simulink model "UAV_GuidanceWaypointScenario"  (R2026a)
settings: Solver=ode45  StopTime=60  MaxStep=0.01
PreLoadFcn:
  | setup_uav_scenario;  % scene must exist before the Scenario blocks initialise on load
InitFcn:
  | setup_uav_scenario;  % recreate the uavScenario handle object before each run
model workspace (MAT data in the model file):
  ctrl.mass = 0.1
  ctrl.g = 9.81
  ctrl.Kp_pos = 0.8
  ctrl.vMaxXY = 3
  ctrl.vMaxZ = 1.5
  ctrl.Kv = 2
  ctrl.tiltMax = 0.35
  ctrl.thrustMax = 2
  ctrl.Kyaw = 2
  ctrl.yawRateMax = 1
  gravityNED = 9.81
  hoverThrust = 0.981
  lookaheadDist = 3
  transitionRadius = 1.5
  uavMass = 0.1
  waypoints = [0  0  -5; 20  0  -5; 20  20  -5; 0  20  -5; 0  0  -5]
values from neighbouring files (symbols this model uses):
  lidarSampleTime = 0.1    [setup_uav_scenario.m]
  scenarioSampleTime = 0.1    [setup_uav_scenario.m]
undefined symbols (not defined in the file or in its folder): Lidar, UAV
libraries: uavsimlib x4, uavalgslib x2, robotcorelib x1
settings Model: Creator=PattarapolSangaroon  LastModifiedBy=PattarapolSangaroon

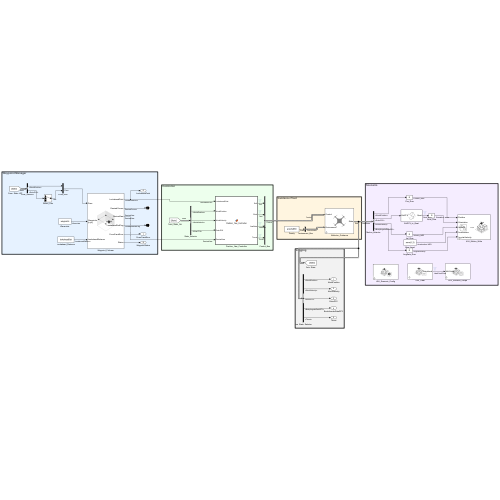
[thumbnail: Simulink's stored preview of the top-level diagram]
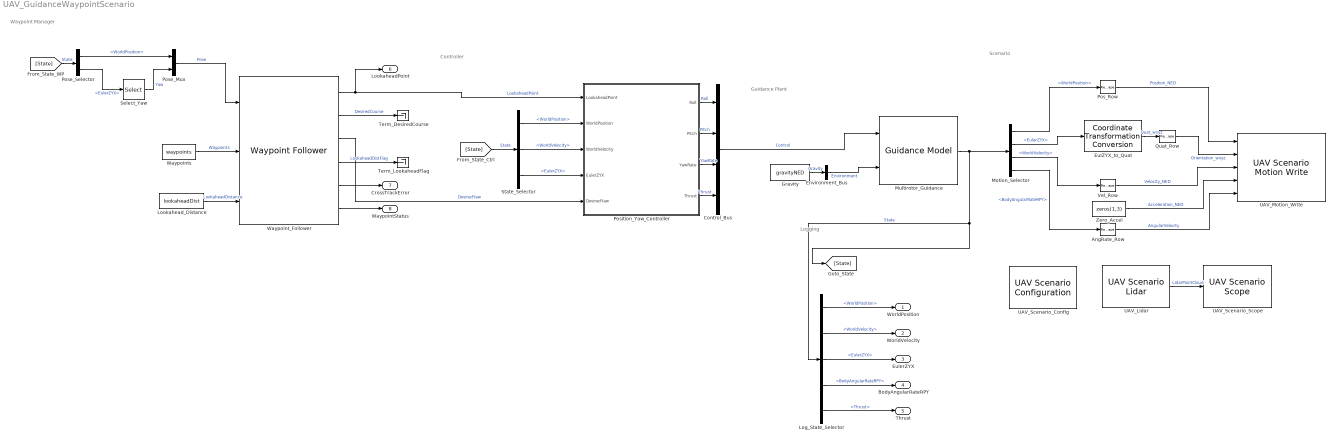
== system UAV_GuidanceWaypointScenario ==
  note: Waypoint Manager
  note: Controller
  note: Guidance Plant
  note: Scenario
  note: Logging
  AngRate_Row : Reshape  OutputDimensionality=Customize  OutputDimensions=[1 3]
  Control_Bus : BusCreator  Inputs=4  OutDataTypeStr=Bus: MultirotorGuidanceControlBus  NonVirtualBus=on
  Environment_Bus : BusCreator  Inputs=1  OutDataTypeStr=Bus: MultirotorGuidanceEnvironmentBus  NonVirtualBus=on
  EulZYX_to_Quat : robotcorelib/Coordinate Transformation Conversion  InputRepresentation=Euler Angles  InputEulerSequence=ZYX  ShowTrVecInputPort=on  OutputRepresentation=Quaternion  OutputEulerSequence=ZYX  ShowTrVecOutputPort=on  SimulateUsing=Code generation
      settings: LibrarySourceBlock=uavutilslib/Coordinate Transformation Conversion
  Gravity : Constant  Value=gravityNED
  Log_State_Selector : BusSelector  OutputSignals=WorldPosition,WorldVelocity,EulerZYX,BodyAngularRateRPY,Thrust
  Lookahead_Distance : Constant  Value=lookaheadDist
  Motion_Selector : BusSelector  OutputSignals=WorldPosition,EulerZYX,WorldVelocity,BodyAngularRateRPY
  Multirotor_Guidance : uavalgslib/Guidance Model  ModelType=MultirotorGuidance  NumInstances=1  SpecifiedDataType=double  SimulateUsing=Code generation  InitialWorldPositionMultirotor=[0; 0; 0]  InitialWorldVelocityMultirotor=[0; 0; 0]  InitialEulerZYXMultirotor=[0; 0; 0]  InitialBodyAngularRateRPYMultirotor=[0; 0; 0]  InitialThrustMultirotor=hoverThrust  InitialNorthFixedWing=0  InitialEastFixedWing=0  InitialHeightFixedWing=0  InitialAirSpeedFixedWing=0  InitialHeadingAngleFixedWing=0  InitialFlightPathAngleFixedWing=0  InitialRollAngleFixedWing=0  InitialRollAngleRateFixedWing=0  PDRollMultirotor=[3402.97,116.67]  PDPitchMultirotor=[3402.97, 116.67]  PYawRateMultirotor=1950  PThrustMultirotor=3900  MassMultirotor=uavMass  PHeightFixedWing=3.9  PHeadingAngleFixedWing=3.9  PFlightPathAngleFixedWing=39  PDRollFixedWing=[3402.97, 116.67]  PAirSpeedFixedWing=1  FlightPathAngleLimitsFixedWing=[-pi/2, pi/2]  StateBusName='MultirotorGuidanceStateBus'  ControlBusName='MultirotorGuidanceControlBus'  EnvironmentBusName='MultirotorGuidanceEnvironmentBus'  DataType=double
  Pos_Row : Reshape  OutputDimensionality=Customize  OutputDimensions=[1 3]
  Pose_Mux : Mux  Inputs=2
  Pose_Selector : BusSelector  OutputSignals=WorldPosition,EulerZYX
  Position_Yaw_Controller : MATLAB Function  TreatAsAtomicUnit=on
  Quat_Row : Reshape  OutputDimensionality=Customize  OutputDimensions=[1 4]
  Select_Yaw : Selector  InputPortWidth=3  IndexOptions=Index vector (dialog)  Indices=1  OutputSizes=1
  State_Selector : BusSelector  OutputSignals=WorldPosition,WorldVelocity,EulerZYX
  Term_DesiredCourse : Terminator
  Term_LookaheadFlag : Terminator
  UAV_Lidar : uavsimlib/UAV Scenario Lidar  Priority=3  SensorName=UAV/Lidar  MaxRange=30  RangeAccuracy=0.02  AzimuthLimits=[-180 180]  AzimuthResolution=2  ElevationLimits=[-20 20]  ElevationResolution=2  HasNoise=off  HasOrganizedOutput=off  SampleTime=lidarSampleTime
  UAV_Motion_Write : uavsimlib/UAV Scenario Motion Write  Priority=2  PlatName='UAV'  ReferenceFrame=NED
  UAV_Scenario_Config : uavsimlib/UAV Scenario Configuration  Priority=1  UAVScenarioObject=uavScene  SampleTime=scenarioSampleTime  UpdateParam=false  SensorMotionBusName='SensorMotionBus'  PlatformMotionBusName='PlatformMotionBus'  ScenarioMotionBusName='ScenarioMotionBus'  ScenarioMotionSignalName='ScenarioMotions'
  UAV_Scenario_Scope : uavsimlib/UAV Scenario Scope  Priority=4  SensorNameTable={'UAV/Lidar','on'}  SampleTime=lidarSampleTime
  Vel_Row : Reshape  OutputDimensionality=Customize  OutputDimensions=[1 3]
  Waypoint_Follower : uavalgslib/Waypoint Follower  UAVType=multirotor  StartFrom=first  TransitionRadiusSource=internal  TransitionRadius=transitionRadius  MinLookaheadDistance=0.1  HoverAtLastWaypoint=on  InterpolateYaw=on  YawInput=off  ShowCrossTrackErrorOutput=on  ShowStatusOutput=on  ShowWaypointIndexOutput=off  SimulateUsing=Code generation
  Waypoints : Constant  Value=waypoints
  Zero_Accel : Constant  Value=zeros(1,3)
  WorldPosition : Outport
  WorldVelocity : Outport  Port=2
  EulerZYX : Outport  Port=3
  BodyAngularRateRPY : Outport  Port=4
  Thrust : Outport  Port=5
  LookaheadPoint : Outport  Port=6
  CrossTrackError : Outport  Port=7
  WaypointStatus : Outport  Port=8
  wires:
  Log_State_Selector/4 -> BodyAngularRateRPY/1  "<BodyAngularRateRPY>"
  Log_State_Selector/3 -> EulerZYX/1  "<EulerZYX>"
  Log_State_Selector/2 -> WorldVelocity/1  "<WorldVelocity>"
  Log_State_Selector/1 -> WorldPosition/1  "<WorldPosition>"
  Log_State_Selector/5 -> Thrust/1  "<Thrust>"
  [State] -> Pose_Selector/1  "State"
  Pose_Selector/1 -> Pose_Mux/1  "<WorldPosition>"
  Pose_Selector/2 -> Select_Yaw/1  "<EulerZYX>"
  Select_Yaw/1 -> Pose_Mux/2  "Yaw"
  Pose_Mux/1 -> Waypoint_Follower/1  "Pose"
  Waypoints/1 -> Waypoint_Follower/2  "Waypoints"
  Lookahead_Distance/1 -> Waypoint_Follower/3  "LookaheadDistance"
  Waypoint_Follower/1 -> Position_Yaw_Controller/1(LookaheadPoint), LookaheadPoint/1  "LookaheadPoint"
  Waypoint_Follower/2 -> Term_DesiredCourse/1  "DesiredCourse"
  Waypoint_Follower/3 -> Position_Yaw_Controller/5(DesiredYaw)  "DesiredYaw"
  Waypoint_Follower/4 -> Term_LookaheadFlag/1  "LookaheadDistFlag"
  Waypoint_Follower/5 -> CrossTrackError/1
  Waypoint_Follower/6 -> WaypointStatus/1
  [State] -> State_Selector/1  "State"
  State_Selector/1 -> Position_Yaw_Controller/2(WorldPosition)  "<WorldPosition>"
  State_Selector/2 -> Position_Yaw_Controller/3(WorldVelocity)  "<WorldVelocity>"
  State_Selector/3 -> Position_Yaw_Controller/4(EulerZYX)  "<EulerZYX>"
  Position_Yaw_Controller/1(Roll) -> Control_Bus/1  "Roll"
  Position_Yaw_Controller/2(Pitch) -> Control_Bus/2  "Pitch"
  Position_Yaw_Controller/3(YawRate) -> Control_Bus/3  "YawRate"
  Position_Yaw_Controller/4(Thrust) -> Control_Bus/4  "Thrust"
  Control_Bus/1 -> Multirotor_Guidance/1  "Control"
  Gravity/1 -> Environment_Bus/1  "Gravity"
  Environment_Bus/1 -> Multirotor_Guidance/2  "Environment"
  Multirotor_Guidance/1 -> [State], Log_State_Selector/1, Motion_Selector/1  "State"
  Motion_Selector/1 -> Pos_Row/1  "<WorldPosition>"
  Motion_Selector/2 -> EulZYX_to_Quat/1  "<EulerZYX>"
  EulZYX_to_Quat/1 -> Quat_Row/1  "Quat_wxyz"
  Motion_Selector/3 -> Vel_Row/1  "<WorldVelocity>"
  Motion_Selector/4 -> AngRate_Row/1  "<BodyAngularRateRPY>"
  Pos_Row/1 -> UAV_Motion_Write/1  "Position_NED"
  Quat_Row/1 -> UAV_Motion_Write/2  "Orientation_wxyz"
  Vel_Row/1 -> UAV_Motion_Write/3  "Velocity_NED"
  Zero_Accel/1 -> UAV_Motion_Write/4  "Acceleration_NED"
  AngRate_Row/1 -> UAV_Motion_Write/5  "AngularVelocity"
  UAV_Lidar/1 -> UAV_Scenario_Scope/1  "LidarPointCloud"

== matlab function UAV_GuidanceWaypointScenario/Position_Yaw_Controller ==
  data: LookaheadPoint input; Roll output; WorldPosition input; WorldVelocity input; EulerZYX input; DesiredYaw input; Pitch output; YawRate output; Thrust output; ctrl parameter
function [Roll, Pitch, YawRate, Thrust] = Position_Yaw_Controller(LookaheadPoint, WorldPosition, WorldVelocity, EulerZYX, DesiredYaw, ctrl)
%#codegen
% Waypoint tracking controller for the multirotor Guidance Model.
% Source of the MATLAB Function block in UAV_GuidanceWaypointFollowing.slx.
% Frame: NED [north east down]. EulerZYX = [yaw pitch roll].
% Small-angle Guidance Model kinematics (consistent with the step tests:
% +roll -> +east, +pitch -> -north):
%   aN = -g*(pitch*cos(yaw) + roll*sin(yaw))
%   aE = -g*(pitch*sin(yaw) - roll*cos(yaw))
%   aD =  g - Thrust*cos(roll)*cos(pitch)/mass

yaw = EulerZYX(1);

% Outer loop: position error -> velocity command (with limits)
vCmd = ctrl.Kp_pos * (LookaheadPoint(:) - WorldPosition(:));
speedXY = norm(vCmd(1:2));
if speedXY > ctrl.vMaxXY
    vCmd(1:2) = vCmd(1:2) * (ctrl.vMaxXY / speedXY);
end
vCmd(3) = min(max(vCmd(3), -ctrl.vMaxZ), ctrl.vMaxZ);

% Inner loop: velocity error -> acceleration command (NED)
aCmd = ctrl.Kv * (vCmd - WorldVelocity(:));

% Rotate horizontal acceleration into the heading frame
aFwd   =  cos(yaw)*aCmd(1) + sin(yaw)*aCmd(2);
aRight = -sin(yaw)*aCmd(1) + cos(yaw)*aCmd(2);

% Acceleration -> attitude and thrust
Pitch = min(max(-aFwd   / ctrl.g, -ctrl.tiltMax), ctrl.tiltMax);
Roll  = min(max( aRight / ctrl.g, -ctrl.tiltMax), ctrl.tiltMax);
Thrust = ctrl.mass * (ctrl.g - aCmd(3)) / (cos(Roll) * cos(Pitch));
Thrust = min(max(Thrust, 0), ctrl.thrustMax);

% Yaw: wrapped heading error -> yaw-rate command
yawErr = atan2(sin(DesiredYaw - yaw), cos(DesiredYaw - yaw));
YawRate = min(max(ctrl.Kyaw * yawErr, -ctrl.yawRateMax), ctrl.yawRateMax);
end
